simulink model "PMSM_DQ_MIL"  (R2024a)
settings: Solver=ode4  StartTime=0.0  StopTime=0.1  FixedStep=0.0000125  RelTol=1e-3
settings Model: Creator=ASUS  LastModifiedBy=ASUS

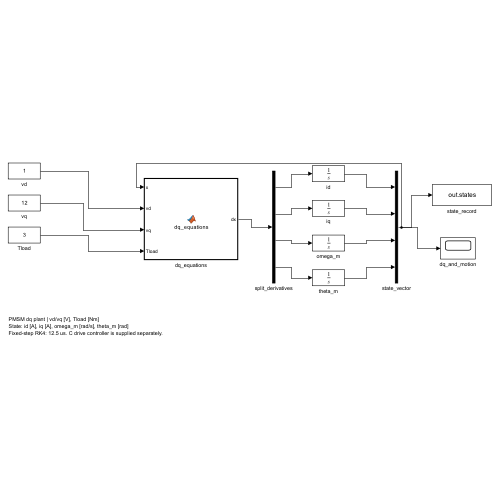
[thumbnail: Simulink's stored preview of the top-level diagram]
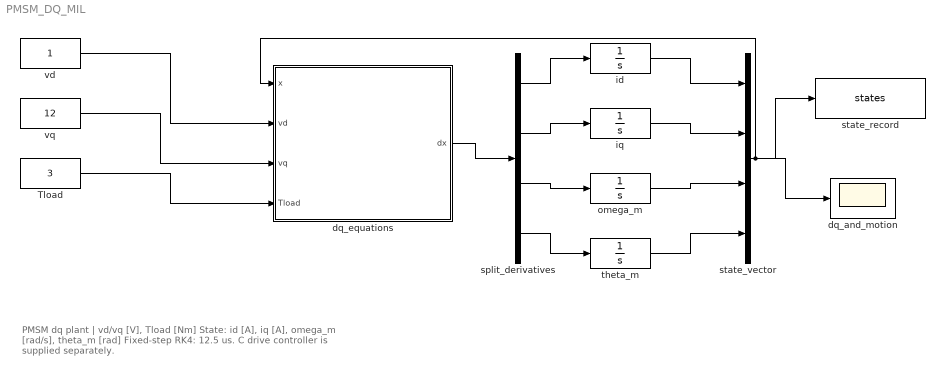
== system PMSM_DQ_MIL ==
  note: PMSM dq plant | vd/vq [V], Tload [Nm]
      | State: id [A], iq [A], omega_m [rad/s], theta_m [rad]
      | Fixed-step RK4: 12.5 us. C drive controller is supplied separately.
  Tload : Constant  Value=3
  dq_and_motion : Scope
  dq_equations : MATLAB Function  TreatAsAtomicUnit=on
  id : Integrator
  iq : Integrator
  omega_m : Integrator
  split_derivatives : Demux
  state_record : ToWorkspace  VariableName=states  SaveFormat=Structure With Time  SampleTime=-1
  state_vector : Mux
  theta_m : Integrator
  vd : Constant
  vq : Constant  Value=12
  wires:
  split_derivatives/1 -> id/1
  id/1 -> state_vector/1
  split_derivatives/2 -> iq/1
  iq/1 -> state_vector/2
  split_derivatives/3 -> omega_m/1
  omega_m/1 -> state_vector/3
  split_derivatives/4 -> theta_m/1
  theta_m/1 -> state_vector/4
  state_vector/1 -> dq_equations/1(x), state_record/1, dq_and_motion/1
  vd/1 -> dq_equations/2(vd)
  vq/1 -> dq_equations/3(vq)
  Tload/1 -> dq_equations/4(Tload)
  dq_equations/1(dx) -> split_derivatives/1

== matlab function PMSM_DQ_MIL/dq_equations ==
  data: x input; dx output; vd input; vq input; Tload input
function dx = dq_equations(x,vd,vq,Tload)
% PMSM in rotor dq coordinates; SI inputs and states.
Rs=0.12; Ld=0.0004; Lq=0.0008; flux=0.085; J=0.006; B=0.001; pairs=4;
id=x(1); iq=x(2); omega=x(3); we=pairs*omega;
Te=1.5*pairs*(flux+(Ld-Lq)*id)*iq;
opposing=Tload*omega/sqrt(omega*omega+0.04);
dx=[(vd-Rs*id+we*Lq*iq)/Ld; (vq-Rs*iq-we*(Ld*id+flux))/Lq;
 (Te-opposing-B*omega)/J; omega];
end
